simulink model "linear_numerical_model"  (R2024b)
settings: Solver=ode4  StartTime=0.0  StopTime=150  FixedStep=0.001  RelTol=1e-3
PreLoadFcn:
  | load linsys1.mat
  | load op_trim3.mat
undefined symbols (not defined in the file or in its folder): linsys1, op_trim3
settings Model: Creator=LocoalKOH  LastModifiedBy=LocoalKOH

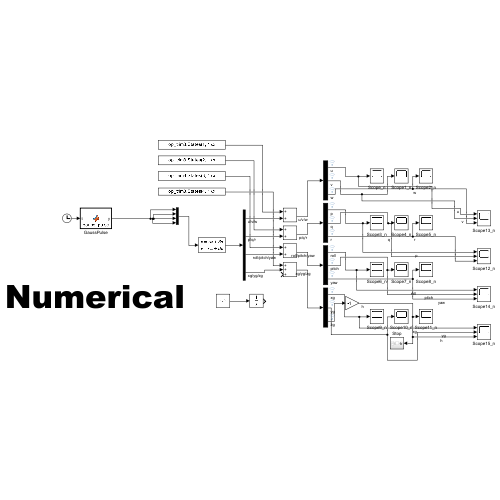
[thumbnail: Simulink's stored preview of the top-level diagram]
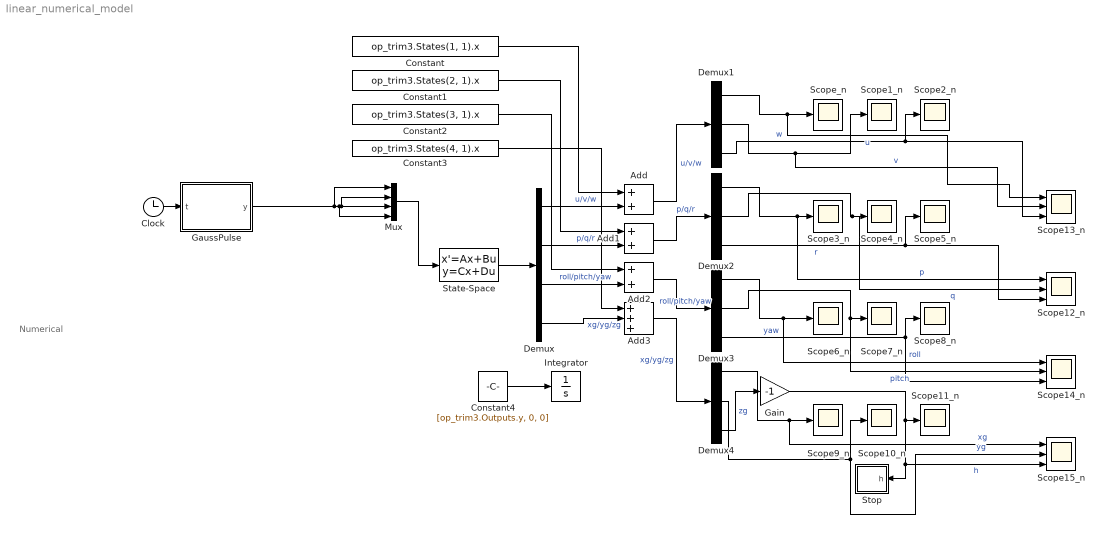
== system linear_numerical_model ==
  note: Numerical
  Add : Sum
  Add1 : Sum
  Add2 : Sum
  Add3 : Sum  Inputs=+++
  Clock : Clock
  Constant : Constant  Value=op_trim3.States(1, 1).x
  Constant1 : Constant  Value=op_trim3.States(2, 1).x
  Constant2 : Constant  Value=op_trim3.States(3, 1).x
  Constant3 : Constant  Value=op_trim3.States(4, 1).x
  Constant4 : Constant  Value=[op_trim3.Outputs.y, 0, 0]
  Demux : Demux
  Demux{1..4} (4 alike) : Demux  Outputs=3
  Gain : Gain  Gain=-1
  GaussPulse : MATLAB Function  TreatAsAtomicUnit=on
  Integrator : Integrator
  Mux : Mux
  Scope10_n : Scope
  Scope11_n : Scope
  Scope12_n : Scope  NumInputPorts=3
  Scope13_n : Scope  NumInputPorts=3
  Scope14_n : Scope  NumInputPorts=3
  Scope15_n : Scope  NumInputPorts=3
  Scope1_n : Scope
  Scope2_n : Scope
  Scope3_n : Scope
  Scope4_n : Scope
  Scope5_n : Scope
  Scope6_n : Scope
  Scope7_n : Scope
  Scope8_n : Scope
  Scope9_n : Scope
  Scope_n : Scope
  State-Space : StateSpace  A=linsys1.A  B=linsys1.B  C=linsys1.C  D=linsys1.D  InitialCondition=zeros(12,1)  ContinuousStateAttributes={'u','v','w','p','q','r','roll','pitch','yaw','xg','yg','zg'}
  Stop : Subsystem
  wires:
  Mux/1 -> State-Space/1
  State-Space/1 -> Demux/1
  Add/1 -> Demux1/1  "u/v/w"
  Add1/1 -> Demux2/1  "p/q/r"
  Add2/1 -> Demux3/1  "roll/pitch/yaw"
  Add3/1 -> Demux4/1  "xg/yg/zg"
  Demux/1 -> Add/2  "u/v/w"
  Demux/2 -> Add1/2  "p/q/r"
  Demux/3 -> Add2/2  "roll/pitch/yaw"
  Demux/4 -> Add3/2  "xg/yg/zg"
  Constant3/1 -> Add3/1
  Constant2/1 -> Add2/1
  Constant1/1 -> Add1/1
  Constant/1 -> Add/1
  Demux1/1 -> Scope13_n/1, Scope_n/1  "u"
  Demux1/2 -> Scope13_n/2, Scope1_n/1  "v"
  Demux1/3 -> Scope13_n/3, Scope2_n/1  "w"
  Demux2/1 -> Scope12_n/1, Scope3_n/1  "p"
  Demux2/2 -> Scope12_n/2, Scope4_n/1  "q"
  Demux2/3 -> Scope12_n/3, Scope5_n/1  "r"
  Demux3/1 -> Scope14_n/1, Scope6_n/1  "roll"
  Demux3/2 -> Scope14_n/2, Scope7_n/1  "pitch"
  Demux3/3 -> Scope14_n/3, Scope8_n/1  "yaw"
  Demux4/1 -> Scope15_n/1, Scope9_n/1  "xg"
  Demux4/2 -> Scope15_n/2, Scope10_n/1  "yg"
  Demux4/3 -> Gain/1  "zg"
  Gain/1 -> Scope11_n/1, Scope15_n/3, Stop/1(h)  "h"
  Constant4/1 -> Integrator/1
  Clock/1 -> GaussPulse/1(t)
  GaussPulse/1(y) -> Mux/1, Mux/4, Mux/2, Mux/3

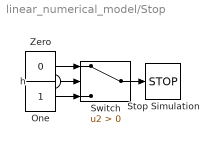
== system linear_numerical_model/Stop ==
  h : Inport
  One : Constant  OutDataTypeStr=Inherit: Inherit via back propagation
  Stop Simulation : Stop
  Switch : Switch  Criteria=u2 > Threshold  SaturateOnIntegerOverflow=off  InputSameDT=off
  Zero : Constant  Value=0  OutDataTypeStr=Inherit: Inherit via back propagation
  wires:
  One/1 -> Switch/3
  Zero/1 -> Switch/1
  Switch/1 -> Stop Simulation/1
  h/1 -> Switch/2

== matlab function linear_numerical_model/GaussPulse ==
  data: t input; y output
function y = gauss_pulse(t)
    y = 0.1 * exp(-(t - 5)^2 / 0.1);  % 在t=5秒附近有扰动
end
